simulink model "s20260910_config2torque_sim_chatgpt_multi_torque"  (R2025a)
settings: Solver=daessc  StartTime=0.0  StopTime=20  FixedStep=0.01  MaxStep=0.05  RelTol=1e-3  AbsTol=1e-3  EnableMultiTasking=on
undefined symbols (not defined in the file or in its folder): X, Y, Z
libraries: sm_lib x9, nesl_utility x4, snake_single_module_library_torque x1, slpidlib x1, simulink x1, spsSawtoothGeneratorLib x1, cstblocks x1, snake_single_module_library_torque_multi x1
settings Model: Creator=dperera  LastModifiedBy=dperera
settings SolverCC: AutoScaleAbsTol=off  AlgebraicLoopSolver=TrustRegion  MaxZcPerStep=1.0
settings DataIOCC: LimitDataPoints=on  MaxDataPoints=10000
settings OptimizationCC: ReuseModelBlockBuffer=off  LifeSpan=inf
settings DebuggingCC: UnconnectedInputMsg=warning  UnconnectedOutputMsg=warning  UnconnectedLineMsg=warning  AllowSymbolicDim=off  SubsystemReferenceDiagnosticForUnitTest=warning  SFUnexpectedBacktrackingDiag=warning  SFNoUnconditionalDefaultTransitionDiag=warning  SFExecutionAtInitializationDiag=none  ArithmeticOperatorsInVariantConditions=warning
settings ModelReferenceCC: EnableRefExpFcnMdlSchedulingChecks=on
settings SFSimCC: SimUseLocalCustomCode=off  CustomCodeUndefinedFunction=UseInterfaceOnly
settings RTWCC: RTWUseLocalCustomCode=off  GPUComputeCapability=3.5  DLArmComputeVersion=19.05
settings CodeAppCC: StateflowObjectComments=on
settings GRTTargetCC: TargetLangStandard=C89/C90 (ANSI)
settings ConfigComp: CovMetricSettings=dw  CovSaveCumulativeToWorkspaceVar=on  CovSaveSingleToWorkspaceVar=on  CovExternalEMLEnable=off  CovSFcnEnable=off
settings SimscapeCC: SimscapeLogType=all  SimscapeLogSimulationStatistics=on  SimscapeLogDataHistory=10000.0

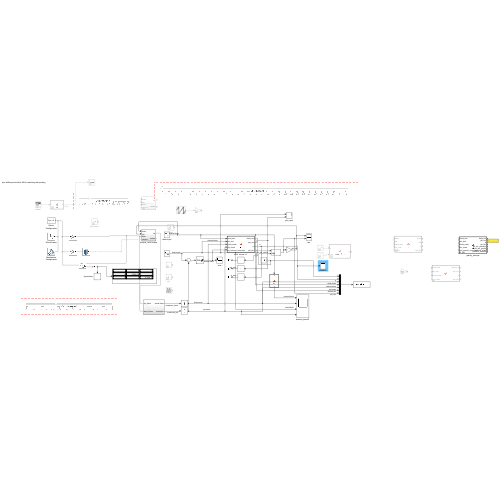
[thumbnail: Simulink's stored preview of the top-level diagram]
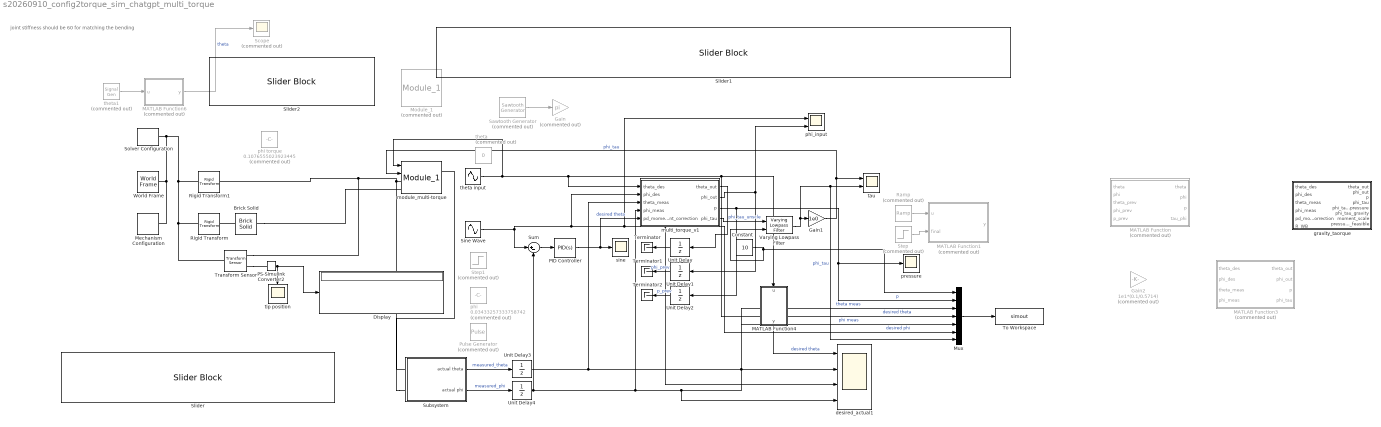
== system s20260910_config2torque_sim_chatgpt_multi_torque ==
  note: joint stiffness should be 60 for matching the bending
  Brick Solid : sm_lib/Body Elements/Brick Solid  BrickDimensions=[0.5 0.5 0.01]  BrickDimensionsUnits=m  ExportEntireGeometry=on  InertiaType=CalculateFromGeometry  BasedOnType=Density  Density=1000  DensityUnits=kg/m^3  Mass=1  MassUnits=kg  CenterOfMass=[0 0 0]  CenterOfMassUnits=m  MomentsOfInertia=[1 1 1]  MomentsOfInertiaUnits=kg*m^2  ProductsOfInertia=[0 0 0]  ProductsOfInertiaUnits=kg*m^2  GraphicType=FromGeometry  MarkerShape=Sphere  MarkerSize=10  GraphicVisPropType=SimpleVisualProperties  GraphicDiffuseColor=[0.5 0.5 0.5]  GraphicOpacity=1  GraphicSpecularColor=[0.5 0.5 0.5 1.0]  GraphicAmbientColor=[0.15 0.15 0.15 1.0]  GraphicEmissiveColor=[0.0 0.0 0.0 1.0]  GraphicShininess=75  DoExposeReferenceFrame=on  SerializedFrames=<Frames/>
  Constant : Constant  Value=10
  Display : Display
  Gain : Gain  Commented=on  Gain=pi
  Gain1 : Gain  Gain=1e0
  Gain2 : Gain  Commented=on  Gain=1e1*(0.1/0.5714)
  MATLAB Function : MATLAB Function  Commented=on  TreatAsAtomicUnit=on
  MATLAB Function1 : MATLAB Function  Commented=on  TreatAsAtomicUnit=on
  MATLAB Function3 : MATLAB Function  Commented=on  TreatAsAtomicUnit=on
  MATLAB Function4 : MATLAB Function  TreatAsAtomicUnit=on
  MATLAB Function6 : MATLAB Function  Commented=on  TreatAsAtomicUnit=on
  Mechanism Configuration : sm_lib/Utilities/Mechanism Configuration  UniformGravity=Constant  GravityVector=[0 0 -9.80665]  GravityVectorUnits=m/s^2  LinearizationDelta=0.001  JointModeTransitionNonlinearIterations=2
  Module_1 : snake_single_module_library_torque/Module_1  Commented=on  SystemSampleTime=-1  VariantActivationTime=update diagram  EmptyChoice=off  PassThrough=off  PassThroughVariantControl=(default)  EmptyChoiceVariantControl=(default)  AllowFlexibleInterface=on  Latency=0  AutoFrameSizeCalculation=off
  Mux : Mux  Inputs=7
  PID Controller : slpidlib/PID Controller  Controller=PID  Form=Parallel  TimeDomain=Continuous-time  UseExternalTs=off  SampleTime=-1  IntegratorMethod=Forward Euler  FilterMethod=Forward Euler  ControllerParametersSource=internal  P=0.3  I=0.1  UseKiTs=off  D=0.0001  UseExternalDerivativeSource=off  N=100  UseFilter=on  TunerSelectOption=Frequency Response Based  InitialConditionSource=internal  InitialConditionForIntegrator=0  InitialConditionForFilter=0  DifferentiatorICPrevScaledInput=0  ExternalReset=none  TrackingMode=off  Kt=1  LimitOutput=on  SatLimitsSource=internal  UpperSaturationLimit=inf  LowerSaturationLimit=-inf  LinearizeAsGain=on  AntiWindupMode=back-calculation  Kb=1  LimitIntegrator=off  UpperIntegratorSaturationLimit=inf  LowerIntegratorSaturationLimit=-inf  POutMin=[]  POutMax=[]  IOutMin=[]  IOutMax=[]  DOutMin=[]  DOutMax=[]  NOutMin=[]  NOutMax=[]  SumOutMin=[]  SumOutMax=[]  SaturationOutMin=[]  SaturationOutMax=[]  PParamMin=[]  PParamMax=[]  IParamMin=[]  IParamMax=[]  DParamMin=[]  DParamMax=[]  NParamMin=[]  NParamMax=[]  KbParamMin=[]  KbParamMax=[]  KtParamMin=[]  KtParamMax=[]  KbOutMin=[]  KbOutMax=[]  KtOutMin=[]  KtOutMax=[]  IntegratorOutMin=[]  IntegratorOutMax=[]  FilterOutMin=[]  FilterOutMax=[]  SumI1OutMin=[]  SumI1OutMax=[]  SumI2OutMin=[]  SumI2OutMax=[]  SumI3OutMin=[]  SumI3OutMax=[]  SumI4OutMin=[]  SumI4OutMax=[]  SumDOutMin=[]  SumDOutMax=[]  DifferentiatorOutMin=[]  DifferentiatorOutMax=[]  FilterDiffOutCoefMin=[]  FilterDiffOutCoefMax=[]  ReciprocalOutMin=[]  ReciprocalOutMax=[]  SumDenOutMin=[]  SumDenOutMax=[]  SumNumOutMin=[]  SumNumOutMax=[]  DivideOutMin=[]  DivideOutMax=[]  UdiffTsProdOutMin=[]  UdiffTsProdOutMax=[]  NTsProdOutMin=[]  NTsProdOutMax=[]  UintegralTsProdOutMin=[]  UintegralTsProdOutMax=[]  UngainTsProdOutMin=[]  UngainTsProdOutMax=[]  ClampingZeroOutDataTypeStr=Inherit: Inherit via back propagation  ClampingZeroOutMin=[]  ClampingZeroOutMax=[]  FilterDenConstantOutDataTypeStr=Inherit: Inherit via back propagation  FilterDenConstantOutMin=[]  FilterDenConstantOutMax=[]  PCopyOutDataTypeStr=Inherit: Inherit via back propagation  PCopyOutMin=[]  PCopyOutMax=[]  NCopyOutDataTypeStr=Inherit: Inherit via back propagation  NCopyOutMin=[]  NCopyOutMax=[]  IntegratorContinuousStateAttributes=''  IntegratorStateMustResolveToSignalObject=off  IntegratorRTWStateStorageClass=Auto  FilterContinuousStateAttributes=''  FilterStateMustResolveToSignalObject=off  FilterRTWStateStorageClass=Auto  ParallelPVariant=InternalParameters  IdealPVariant=Disabled  IVariant=InternalParameters  DVariant=InternalParameters  IntegratorVariant=Continuous  SatVariant=Enabled  AWVariant=BackCalculation  PCopyVariant=Disabled  TRVariant=Disabled  FdbkBlocksVariant=Forward  IdealPFdbkVariant=Disabled  SatFdbkVariant=Disabled  DerivativeFilterVariant=ContFilter  NVariant=InternalParameters  NCopyVariant=Disabled  FilterICVariant=InternalICsFilter  IntegratorICVariant=InternalICs  ExternalResetVariant=Disabled  TRSumVariant=Passthrough  SumFdbkVariant=Disabled  SumVariant=Sum_PID  TsampFilterVariant=InternalTs  TsampNgainVariant=Passthrough  TsampIntegralVariant=Disabled_SignalSpec  ExternalSaturationOutDataTypeStr=Inherit: Same as second input  DerivativeSourceVariant=ErrorSignal  PreIntVariant=InternalPreInt
  PS-Simulink Converter2 : nesl_utility/PS-Simulink Converter  PhysicalDomain=network_engine_domain  SubClassName=ps_output  LeftPortType=input  RightPortType=output  PseudoPeriodic=off  Frequencies=[]  VectorFormat=inherit  Unit=inherit  AffineConversion=off
  Pulse Generator : DiscretePulseGenerator  Commented=on  PulseType=Time based  Amplitude=pi/3  Period=4  PulseWidth=50  PhaseDelay=1
  Ramp : simulink/Sources/Ramp  Commented=on  slope=0.01*2*pi  start=1  InitialOutput=0.001
  Rigid Transform : sm_lib/Frames and Transforms/Rigid Transform  RotationMethod=None  FollAlignAxisA=+X  BaseAlignAxisA=+Y  FollAlignAxisB=+Y  BaseAlignAxisB=+Z  RotationStandardAxis=+Z  RotationAngle=0  RotationAngleUnits=deg  RotationArbitraryAxis=[0 0 1]  RotationSequenceAxes=FollowerAxes  RotationSequence=XYX  RotationSequenceAngles=[0 0 0]  RotationSequenceAnglesUnits=deg  RotationMatrix=[1 0 0;0 1 0;0 0 1]  Quaternion=[1 0 0 0]  TranslationMethod=StandardAxis  TranslationCartesianOffset=[0 0 0]  TranslationCartesianOffsetUnits=m  TranslationStandardAxis=+Z  TranslationStandardOffset=-0.03  TranslationStandardOffsetUnits=m  TranslationROffset=0  TranslationROffsetUnits=m  TranslationThetaOffset=0  TranslationThetaOffsetUnits=deg  TranslationZOffset=0  TranslationZOffsetUnits=m
  Rigid Transform1 : sm_lib/Frames and Transforms/Rigid Transform  RotationMethod=StandardAxis  FollAlignAxisA=+X  BaseAlignAxisA=+Y  FollAlignAxisB=+Y  BaseAlignAxisB=+Z  RotationStandardAxis=+X  RotationAngle=pi/2  RotationAngleUnits=rad  RotationArbitraryAxis=[0 0 1]  RotationSequenceAxes=FollowerAxes  RotationSequence=XYX  RotationSequenceAngles=[0 0 0]  RotationSequenceAnglesUnits=deg  RotationMatrix=[1 0 0;0 1 0;0 0 1]  Quaternion=[1 0 0 0]  TranslationMethod=StandardAxis  TranslationCartesianOffset=[0 0 0]  TranslationCartesianOffsetUnits=m  TranslationStandardAxis=+Z  TranslationStandardOffset=0.5  TranslationStandardOffsetUnits=m  TranslationROffset=0  TranslationROffsetUnits=m  TranslationThetaOffset=0  TranslationThetaOffsetUnits=deg  TranslationZOffset=0  TranslationZOffsetUnits=m
  Sawtooth Generator : spsSawtoothGeneratorLib/Sawtooth Generator  Commented=on  Freq=0.5  Phase=180  Ts=0.001
  Scope : Scope  Commented=on
      settings: ActiveDisplayYMinimum=-3.3334127281449564  ActiveDisplayYMaximum=3.1584952199962761
  Sine Wave : Sin  Amplitude=pi/2-0.3  Bias=pi/2-0.3  Phase=3*pi/2  SampleTime=0
  Slider : SliderBlock  ScaleMin=-3.14  ScaleMax=6
  Slider1 : SliderBlock  ScaleMax=3.14
  Slider2 : SliderBlock  ScaleMax=0.5
  Solver Configuration : nesl_utility/Solver Configuration  PhysicalDomain=network_engine_domain  SubClassName=solver  LeftPortType=input  RightPortType=generic  Tones=[]  Harmonics=[]  SimulateNoise=off  Profile=off  UseLocalSampling=off  EnableSwitchedLinearOptims=on  FrequencyDomain=off  UseCCode=off  RelTol=0.001  AbsTol=1e-06  MinStep=1e-09  ToWorkspace=off  RevertToSquareIcSolve=off  NumHomotopyIterations=100  PhasorMode=off  PhasorModeNumHarmonics=1  ConsistencySolver=NEWTON_XTOL_AFTER_FTOL  IndexReductionMethod=DerivativeReplacement  DoDC=off  ResidualTolerance=1e-09  ConsistencyTolSource=GLOBAL  ConsistencyAbsTol=0.001  ConsistencyRelTol=0.001  ConsistencyTolFactor=0.001  UseLocalSolver=off  LocalSolverChoice=NE_BACKWARD_EULER_ADVANCER  ResolveIndetEquations=on  FunctionEvalNumThread=1  LocalSolverSampleTime=0.001  DoFixedCost=off  MaxNonlinIter=3  MaxModeIter=2  ComputeImpulses=off  ImpulseIterations=2  LinearAlgebra=Sparse  LinearAlgebraNumThread=0  EquationFormulation=NE_TIME_EF  DelaysMemoryBudget=1024  AutomaticFiltering=on  FilteringTimeConstant=0.001  PartitionStorageMethod=AS_NEEDED  PartitionMemoryBudget=1024  PartitionMethod=FAST  MultibodyUseLocalSolver=off  MultibodyLocalSolverChoice=ODE1  MultibodyLocalSolverSampleTime=0.001
  Step : Step  Commented=on  Time=2  SampleTime=0
  Step1 : Step  Commented=on  After=pi/3  SampleTime=0
  Subsystem : Subsystem
  Sum : Sum  Inputs=|+-
  Terminator : Terminator
  Terminator1 : Terminator
  Terminator2 : Terminator
  To Workspace : ToWorkspace  VariableName=simout  SaveFormat=Timeseries  SampleTime=-1
      settings: Save2DSignal=2-D array (concatenate along first dimension)
  Transform Sensor : sm_lib/Frames and Transforms/Transform Sensor  MeasurementFrame=World  RotationSequence=XYX  SenseAngle=off  SenseAxis=off  SenseQ=off  SenseR=on  SenseRotationSequence=off  SenseOmegaX=off  SenseOmegaY=off  SenseOmegaZ=off  SenseOmega=off  SenseQDot=off  SenseRDot=off  SenseRotationSequenceDot=off  SenseAlphaX=off  SenseAlphaY=off  SenseAlphaZ=off  SenseAlpha=off  SenseQDDot=off  SenseRDDot=off  SenseX=off  SenseY=off  SenseZ=off  SenseXYZ=off  SenseRad=off  SenseAzim=off  SenseDist=off  SenseInc=off  SenseXDot=off  SenseYDot=off  SenseZDot=off  SenseXYZDot=off  SenseRadDot=off  SenseAzimDot=off  SenseDistDot=off  SenseIncDot=off  SenseXDDot=off  SenseYDDot=off  SenseZDDot=off  SenseXYZDDot=off  SenseRadDDot=off  SenseAzimDDot=off  SenseDistDDot=off  SenseIncDDot=off
  Unit Delay : UnitDelay  InitialCondition=[0]  SampleTime=-1  HasFrameUpgradeWarning=on
  Unit Delay1 : UnitDelay  InitialCondition=0.0001  SampleTime=-1  HasFrameUpgradeWarning=on
  Unit Delay2 : UnitDelay  InitialCondition=[0.0001;0.01;0.001]  SampleTime=-1  HasFrameUpgradeWarning=on
  Unit Delay3 : UnitDelay  InitialCondition=[0]  SampleTime=-1  HasFrameUpgradeWarning=on
  Unit Delay4 : UnitDelay  InitialCondition=0.0001  SampleTime=-1  HasFrameUpgradeWarning=on
  Varying Lowpass Filter : cstblocks/Linear Parameter Varying/Varying Lowpass Filter  N=1
  World Frame : sm_lib/Frames and Transforms/World Frame
  desired_actual1 : Scope  NumInputPorts=4
      settings: ActiveDisplayYMinimum=-0.37614430678155741  ActiveDisplayYMaximum=3.3852987610340177  DataLoggingVariableName=ScopeData7
  gravity_taorque : MATLAB Function  TreatAsAtomicUnit=on
  module_multi-torque : snake_single_module_library_torque_multi/Module_1  SystemSampleTime=-1  VariantActivationTime=update diagram  EmptyChoice=off  PassThrough=off  PassThroughVariantControl=(default)  EmptyChoiceVariantControl=(default)  AllowFlexibleInterface=on  Latency=0  AutoFrameSizeCalculation=off
  multi_torque_v1 : MATLAB Function  TreatAsAtomicUnit=on
  phi : Constant  Commented=on  Value=0.03433257333758742
  phi torque : Constant  Commented=on  Value=0.1076555023923445
  phi_input : Scope  NumInputPorts=2
      settings: ActiveDisplayYMinimum=-0.36834079509334744  ActiveDisplayYMaximum=3.3160671558401278  DataLoggingVariableName=ScopeData3
  pressure : Scope
      settings: ActiveDisplayYMinimum=-30741.22465781157  ActiveDisplayYMaximum=510004.6447710325  DataLoggingVariableName=ScopeData4
  sine : Scope
      settings: ActiveDisplayYMinimum=-0.41740703510045596  ActiveDisplayYMaximum=3.0703490190244911  DataLoggingVariableName=ScopeData2
  tau : Scope  NumInputPorts=2
      settings: ActiveDisplayYMinimum=-0.07521570426510249  ActiveDisplayYMaximum=0.65254070404289077
  theta : Constant  Commented=on  Value=0
  theta input : Sin  Amplitude=pi-0.1  Frequency=0.1  SampleTime=0
  theta1 : SignalGenerator  Commented=on  WaveForm=sawtooth  Amplitude=pi  Frequency=0.1*2*pi  Units=rad/sec  VectorParams1D=off
  tip position : Scope
      settings: ActiveDisplayYMinimum=-1.2500000000000002  ActiveDisplayYMaximum=1.2500000000000004  DataLoggingVariableName=ScopeData5
  wires:
  Sawtooth Generator/1 -> Gain/1
  theta1/1 -> MATLAB Function6/1(u)
  MATLAB Function6/1(y) -> Scope/1  "theta"
  multi_torque_v1/1(theta_out) -> Unit Delay/1
  multi_torque_v1/2(phi_out) -> Unit Delay1/1, phi_input/2
  multi_torque_v1/3(p) -> Mux/2, pressure/1, Unit Delay2/1  "p"
  theta input/1 -> module_multi-torque/1, multi_torque_v1/1(theta_des), Mux/4, MATLAB Function4/1(u)  "desired theta"
  Ramp/1 -> MATLAB Function1/1(u)
  Step/1 -> MATLAB Function1/2(final)
  MATLAB Function4/1(y) -> desired_actual1/1  "desired theta"
  Gain1/1 -> module_multi-torque/2, tau/1  "phi_tau"
  Sine Wave/1 -> multi_torque_v1/2(phi_des), desired_actual1/3, Mux/6, phi_input/1, Sum/1  "desired phi"
  Subsystem/1(actual theta) -> Unit Delay3/1  "measured_theta"
  Subsystem/2(actual phi) -> Unit Delay4/1  "measured_phi"
  Mux/1 -> To Workspace/1
  PID Controller/1 -> multi_torque_v1/5(pd_moment_correction), sine/1  "desired theta"
  Unit Delay/1 -> Terminator/1
  Unit Delay1/1 -> Terminator1/1  "phi_prev"
  Unit Delay2/1 -> Terminator2/1  "p_prev"
  Unit Delay3/1 -> multi_torque_v1/3(theta_meas), Mux/3, desired_actual1/2  "theta meas"
  Unit Delay4/1 -> multi_torque_v1/4(phi_meas), Mux/5, desired_actual1/4, Sum/2  "phi meas"
  Sum/1 -> PID Controller/1
  multi_torque_v1/4(phi_tau) -> Varying Lowpass Filter/1  "phi_tau_unscle"
  Varying Lowpass Filter/1 -> Mux/7, tau/2, Gain1/1  "phi_tau"
  Constant/1 -> Mux/1, Varying Lowpass Filter/2
  PS-Simulink Converter2/1 -> Display/1, tip position/1
  connections:
  World Frame/RConn1 -- Transform Sensor/LConn1 -- Rigid Transform/LConn1 -- Rigid Transform1/LConn1 -- Solver Configuration/RConn1 -- Mechanism Configuration/RConn1
  Brick Solid/RConn1 -- Rigid Transform/RConn1
  Subsystem/LConn2 -- Transform Sensor/RConn1 -- Rigid Transform1/RConn1 -- module_multi-torque/LConn1
  Brick Solid/LConn1 -- module_multi-torque/LConn2
  Subsystem/LConn1 -- module_multi-torque/RConn1
  Transform Sensor/RConn2 -- PS-Simulink Converter2/LConn1

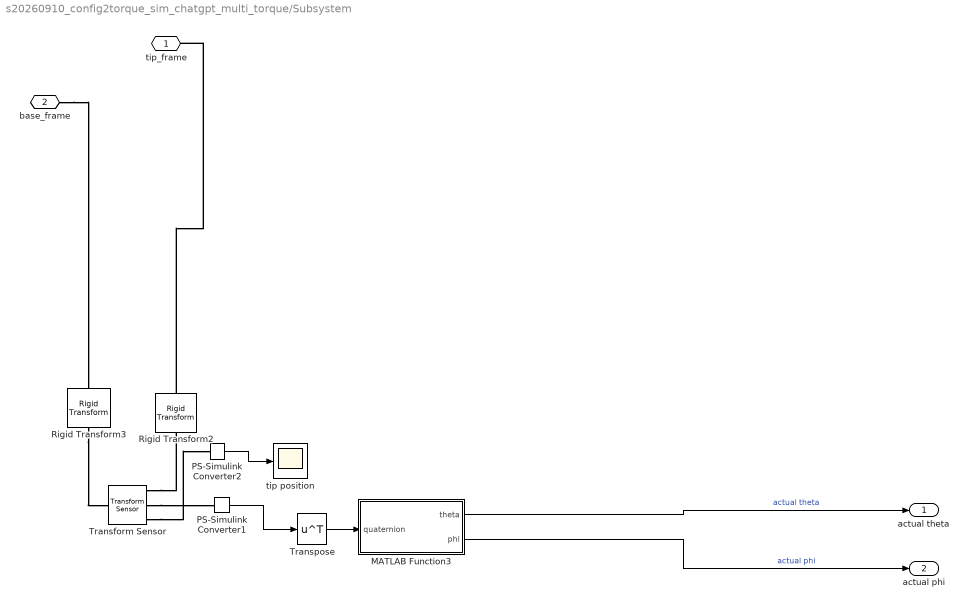
== system s20260910_config2torque_sim_chatgpt_multi_torque/Subsystem ==
  MATLAB Function3 : MATLAB Function  TreatAsAtomicUnit=on
  PS-Simulink Converter1 : nesl_utility/PS-Simulink Converter  PhysicalDomain=network_engine_domain  SubClassName=ps_output  LeftPortType=input  RightPortType=output  PseudoPeriodic=off  Frequencies=[]  VectorFormat=inherit  Unit=inherit  AffineConversion=off
  PS-Simulink Converter2 : nesl_utility/PS-Simulink Converter  PhysicalDomain=network_engine_domain  SubClassName=ps_output  LeftPortType=input  RightPortType=output  PseudoPeriodic=off  Frequencies=[]  VectorFormat=inherit  Unit=inherit  AffineConversion=off
  Rigid Transform2 : sm_lib/Frames and Transforms/Rigid Transform  RotationMethod=RotationSequence  FollAlignAxisA=+X  BaseAlignAxisA=+Y  FollAlignAxisB=+Y  BaseAlignAxisB=+Z  RotationStandardAxis=+Z  RotationAngle=pi  RotationAngleUnits=rad  RotationArbitraryAxis=[0 0 1]  RotationSequenceAxes=FollowerAxes  RotationSequence=XZY  RotationSequenceAngles=[-pi/2 pi 0]  RotationSequenceAnglesUnits=rad  RotationMatrix=[1 0 0;0 1 0;0 0 1]  Quaternion=[1 0 0 0]  TranslationMethod=None  TranslationCartesianOffset=[0 0 0]  TranslationCartesianOffsetUnits=m  TranslationStandardAxis=+Z  TranslationStandardOffset=-0.5  TranslationStandardOffsetUnits=m  TranslationROffset=0  TranslationROffsetUnits=m  TranslationThetaOffset=0  TranslationThetaOffsetUnits=deg  TranslationZOffset=0  TranslationZOffsetUnits=m
  Rigid Transform3 : sm_lib/Frames and Transforms/Rigid Transform  RotationMethod=RotationSequence  FollAlignAxisA=+X  BaseAlignAxisA=+Y  FollAlignAxisB=+Y  BaseAlignAxisB=+Z  RotationStandardAxis=+Z  RotationAngle=pi  RotationAngleUnits=rad  RotationArbitraryAxis=[0 0 1]  RotationSequenceAxes=FollowerAxes  RotationSequence=YXZ  RotationSequenceAngles=[pi -pi/2 0]  RotationSequenceAnglesUnits=rad  RotationMatrix=[1 0 0;0 1 0;0 0 1]  Quaternion=[1 0 0 0]  TranslationMethod=None  TranslationCartesianOffset=[0 0 0]  TranslationCartesianOffsetUnits=m  TranslationStandardAxis=+Z  TranslationStandardOffset=-0.5  TranslationStandardOffsetUnits=m  TranslationROffset=0  TranslationROffsetUnits=m  TranslationThetaOffset=0  TranslationThetaOffsetUnits=deg  TranslationZOffset=0  TranslationZOffsetUnits=m
  Transform Sensor : sm_lib/Frames and Transforms/Transform Sensor  MeasurementFrame=Follower  RotationSequence=XYZ  SenseAngle=off  SenseAxis=off  SenseQ=on  SenseR=off  SenseRotationSequence=off  SenseOmegaX=off  SenseOmegaY=off  SenseOmegaZ=off  SenseOmega=off  SenseQDot=off  SenseRDot=off  SenseRotationSequenceDot=off  SenseAlphaX=off  SenseAlphaY=off  SenseAlphaZ=off  SenseAlpha=off  SenseQDDot=off  SenseRDDot=off  SenseX=off  SenseY=off  SenseZ=off  SenseXYZ=on  SenseRad=off  SenseAzim=off  SenseDist=off  SenseInc=off  SenseXDot=off  SenseYDot=off  SenseZDot=off  SenseXYZDot=off  SenseRadDot=off  SenseAzimDot=off  SenseDistDot=off  SenseIncDot=off  SenseXDDot=off  SenseYDDot=off  SenseZDDot=off  SenseXYZDDot=off  SenseRadDDot=off  SenseAzimDDot=off  SenseDistDDot=off  SenseIncDDot=off
  Transpose : Math  Operator=transpose
  tip position : Scope
      settings: ActiveDisplayYMinimum=-0.036250000065594909  ActiveDisplayYMaximum=0.32625000000729432  DataLoggingVariableName=ScopeData6
  tip_frame : PMIOPort  Side=Left
  base_frame : PMIOPort  Port=2  Side=Left
  actual theta : Outport
  actual phi : Outport  Port=2
  wires:
  PS-Simulink Converter1/1 -> Transpose/1
  Transpose/1 -> MATLAB Function3/1(quaternion)
  MATLAB Function3/2(phi) -> actual phi/1  "actual phi"
  PS-Simulink Converter2/1 -> tip position/1
  MATLAB Function3/1(theta) -> actual theta/1  "actual theta"
  connections:
  Transform Sensor/RConn1 -- Rigid Transform2/RConn1
  Transform Sensor/RConn2 -- PS-Simulink Converter1/LConn1
  Rigid Transform3/RConn1 -- Transform Sensor/LConn1
  Transform Sensor/RConn3 -- PS-Simulink Converter2/LConn1
  base_frame/RConn1 -- Rigid Transform3/LConn1
  Rigid Transform2/LConn1 -- tip_frame/RConn1

== matlab function s20260910_config2torque_sim_chatgpt_multi_torque/MATLAB Function6 ==
  data: u input; y output
function y = fcn(u)

y = wrapToPi(u - pi);

== matlab function s20260910_config2torque_sim_chatgpt_multi_torque/MATLAB Function1 ==
  data: u input; y output; final input
function y = smoothStep(u, final)

y = u*(1-final);

if y <= 0.00001
    y= 0.001;
end

end

== matlab function s20260910_config2torque_sim_chatgpt_multi_torque/MATLAB Function ==
  data: theta input; theta output; phi input; theta_prev input; phi_prev input; p_prev input; phi output; p output; tau_phi output
function [theta, phi, p, tau_phi] = fcn(theta, phi, theta_prev, phi_prev, p_prev)
%#codegen 
% 
% This function computes torque required for the
% 
A = pi * (0.013/2)^2;
r = 0.013;
K = 0.00001;
N = 30;
L = 0.29;
l = L/N;

J_angle = f20260427_3_pressure2config_Jacobian(p_prev, A, K, r);
J_inv = pinv(J_angle);
% p = p_mat(:, i) + J_inv*([theta(i+1); phi(i+1)]-[frw(1,i); frw(2,i)]);
p = p_prev + J_inv*([theta; phi]-[theta_prev; phi_prev]);
% p = m20260427_5_PositivePressures(p);


[f, my, mx, ~, ~] = pressure2force_moment_config(p, A, r, K);
W = [mx; my; 0.0; 0.0; 0.0; f];
J = completeArm_Jacobian(theta_prev, phi_prev, l, N);

tau = J' * W;
tau_phi = tau(2);

== matlab function s20260910_config2torque_sim_chatgpt_multi_torque/gravity_taorque ==
  data: theta_des input; theta_out output; phi_des input; theta_meas input; phi_meas input; phi_out output; p output; phi_tau output; pd_moment_correction input; R_WB input; phi_tau_pressure output; phi_tau_gravity output; moment_scale output; pressure_feasible output
function [theta_out, phi_out, p, phi_tau, ...
          phi_tau_pressure, phi_tau_gravity, ...
          moment_scale, pressure_feasible] = ...
    fcn(theta_des, phi_des, theta_meas, phi_meas, ...
        pd_moment_correction, R_WB)

%#codegen
%
% Inputs:
%   theta_des            : desired bending direction [rad]
%   phi_des              : desired total bending angle [rad]
%   theta_meas           : measured bending direction [rad]
%   phi_meas             : measured total bending angle [rad]
%   pd_moment_correction : PD correction added to bending moment [N*m]
%   R_WB                 : rotation matrix from arm base to world [3x3]
%
%                           v_world = R_WB*v_base
%
% Outputs:
%   theta_out       : desired theta for theta position controller [rad]
%   phi_out         : desired phi for logging [rad]
%   p               : allocated muscle pressures [3x1], Pa
%   phi_tau         : final torque for all 58 phi joints [58x1], N*m
%   phi_tau_pressure: pressure-generated phi-joint torque [58x1], N*m
%   phi_tau_gravity : gravity-compensation torque [58x1], N*m
%   moment_scale    : pressure-allocation moment scaling factor
%   pressure_feasible: true if the requested moment is feasible
%
% phi_tau ordering:
%   phi_tau(1)  = interval 1, Phi1
%   phi_tau(2)  = interval 1, Phi2
%   phi_tau(3)  = interval 2, Phi1
%   phi_tau(4)  = interval 2, Phi2
%   ...
%   phi_tau(57) = interval 29, Phi1
%   phi_tau(58) = interval 29, Phi2

%% Model parameters

A = pi*(0.013/2)^2;     % Effective muscle area [m^2]
r = 0.013;              % Muscle radial offset [m]
K = 0.19223750;         % Continuum bending stiffness [N*m/rad]

N = 29;                 % Number of rigid-link intervals
L = 0.29;               % Arm length [m]
l = L/N;                % Link length [m]

number_phi_joints = 2*N;

% Total module mass is assumed to be 0.100 kg over 30 disks.
% The base disk is fixed but each moving disk retains the same mass.
disk_mass = 0.100/30;   % [kg]

theta_out = theta_des;
phi_out = phi_des;

%% Desired bending moments

% The PD controller modifies the commanded bending moment.
bending_moment_cmd = K*phi_des + pd_moment_correction;

my_des =  bending_moment_cmd*cos(theta_des);
mx_des = -bending_moment_cmd*sin(theta_des);

%% Null-space pressure allocation

Ar = A*r;

% Differential-pressure component. Its sum is zero, so adding a common
% pressure does not change the bending moments.
p_delta = [ ...
    -2*my_des/(3*Ar);
     my_des/(3*Ar) + mx_des/(sqrt(3)*Ar);
     my_des/(3*Ar) - mx_des/(sqrt(3)*Ar)];

p_min = 0;              % Minimum pressure [Pa]
p_max = 350000;         % Maximum pressure: 3.5 bar [Pa]

p_common_min = p_min - min(p_delta);
p_common_max = p_max - max(p_delta);

if p_common_min <= p_common_max

    % Requested bending moment is feasible.
    p_common = 0.5*(p_common_min + p_common_max);

    p = p_delta + p_common;

    moment_scale = 1.0;
    pressure_feasible = true;

else

    % Scale the differential pressures while preserving theta.
    pressure_span = max(p_delta) - min(p_delta);

    if pressure_span > 1e-12
        moment_scale = (p_max - p_min)/pressure_span;
    else
        moment_scale = 1.0;
    end

    p_delta = moment_scale*p_delta;

    p_common_min = p_min - min(p_delta);
    p_common_max = p_max - max(p_delta);

    p_common = 0.5*(p_common_min + p_common_max);

    p = p_delta + p_common;

    pressure_feasible = false;

end

%% Recalculate the achievable moments

moment_y = -(A*r*(-p(2) - p(3) + 2*p(1)))/2;
moment_x =  A*r*sqrt(3)*(p(2) - p(3))/2;

%% Moment-only tip wrench

% Wrench convention:
% [Mx; My; Mz; Fx; Fy; Fz]
%
% The axial force is intentionally excluded.
W_pressure = [moment_x;
              moment_y;
              0;
              0;
              0;
              0];

%% Select the configuration used by the Jacobian and gravity model

% Theta is undefined when the arm is straight. Use commanded theta in
% this small region.
if abs(phi_meas) < 1e-6
    theta_for_J = theta_des;
else
    theta_for_J = theta_meas;
end

phi_for_J = phi_meas;

%% Pressure-generated joint torques

J_tip = completeArm_Jacobian( ...
    theta_for_J, phi_for_J, l, N);

tau_pressure_all = J_tip.'*W_pressure;

phi_tau_pressure = zeros(number_phi_joints,1);

for interval = 1:N

    % Columns in the complete 4N-joint Jacobian
    index_all_phi1 = 4*(interval-1) + 2;
    index_all_phi2 = 4*(interval-1) + 3;

    % Locations in the 2N-element output vector
    index_phi1 = 2*interval - 1;
    index_phi2 = 2*interval;

    phi_tau_pressure(index_phi1) = ...
        tau_pressure_all(index_all_phi1);

    phi_tau_pressure(index_phi2) = ...
        tau_pressure_all(index_all_phi2);
end

%% Convert world gravity into the arm-base frame

gravity_world = [0;
                 0;
                -9.80665];

% R_WB maps base-frame vectors into the world frame.
% Therefore, its transpose maps world vectors into the base frame.
gravity_base = R_WB.'*gravity_world;

gravity_force_disk = disk_mass*gravity_base;

%% Rotation matrices for one rigid-link interval

alpha = phi_for_J/(2*N);

ct = cos(theta_for_J);
st = sin(theta_for_J);

ca = cos(alpha);
sa = sin(alpha);

Rz_theta = [ct, -st, 0;
            st,  ct, 0;
             0,   0, 1];

Rz_minus_theta = [ ct, st, 0;
                   -st, ct, 0;
                     0,  0, 1];

Ry_alpha = [ ca, 0, sa;
              0, 1,  0;
            -sa, 0, ca];

%% Joint axes, joint positions and disk COM positions

joint_axis = zeros(3,number_phi_joints);
joint_position = zeros(3,number_phi_joints);
disk_position = zeros(3,N);

% Pose at the base of the current interval
R_current = eye(3);
position_current = zeros(3,1);

translation_local = [0; 0; l];

for interval = 1:N

    index_phi1 = 2*interval - 1;
    index_phi2 = 2*interval;

    % Apply Rz(theta).
    R_after_theta = R_current*Rz_theta;

    % First phi joint is located at the proximal disk.
    joint_axis(:,index_phi1) = R_after_theta(:,2);
    joint_position(:,index_phi1) = position_current;

    % Apply the first Ry(alpha).
    R_after_phi1 = R_after_theta*Ry_alpha;

    % Translate to the next disk.
    next_disk_position = ...
        position_current + R_after_phi1*translation_local;

    % Second phi joint is located at the distal disk.
    joint_axis(:,index_phi2) = R_after_phi1(:,2);
    joint_position(:,index_phi2) = next_disk_position;

    % Assumption: the disk COM is at the disk-frame origin.
    disk_position(:,interval) = next_disk_position;

    % Complete the interval:
    % Ry(alpha), followed by Rz(-theta).
    R_current = ...
        R_after_phi1*Ry_alpha*Rz_minus_theta;

    position_current = next_disk_position;
end

%% Accumulate downstream gravity forces and moments

% downstream_force(:,i) contains the total gravity force from disk i
% through disk N.
%
% downstream_moment_origin(:,i) contains their total gravity moment
% calculated about the arm-base origin.

downstream_force = zeros(3,N+1);
downstream_moment_origin = zeros(3,N+1);

for disk_number = N:-1:1

    downstream_force(:,disk_number) = ...
        downstream_force(:,disk_number+1) + ...
        gravity_force_disk;

    downstream_moment_origin(:,disk_number) = ...
        downstream_moment_origin(:,disk_number+1) + ...
        cross(disk_position(:,disk_number), ...
              gravity_force_disk);
end

%% Calculate gravity torque at all 58 phi joints

phi_tau_gravity_load = zeros(number_phi_joints,1);

for interval = 1:N

    index_phi1 = 2*interval - 1;
    index_phi2 = 2*interval;

    force_downstream = downstream_force(:,interval);
    moment_downstream_origin = ...
        downstream_moment_origin(:,interval);

    % Gravity moment about the first phi joint
    moment_about_phi1 = ...
        moment_downstream_origin ...
        - cross(joint_position(:,index_phi1), ...
                force_downstream);

    phi_tau_gravity_load(index_phi1) = ...
        joint_axis(:,index_phi1).'*moment_about_phi1;

    % Gravity moment about the second phi joint
    moment_about_phi2 = ...
        moment_downstream_origin ...
        - cross(joint_position(:,index_phi2), ...
                force_downstream);

    phi_tau_gravity_load(index_phi2) = ...
        joint_axis(:,index_phi2).'*moment_about_phi2;
end

%% Gravity compensation

% Gravity compensation acts opposite to the gravity-generated load.
phi_tau_gravity = -phi_tau_gravity_load;

%% Final joint torque commands

% pd_moment_correction is already included in the pressure-generated
% moment. Do not add the same PD output again elsewhere.
phi_tau = phi_tau_pressure + phi_tau_gravity;

end

== matlab function s20260910_config2torque_sim_chatgpt_multi_torque/Subsystem/MATLAB Function3 ==
  data: quaternion input; theta output; phi output
function [theta, phi] = IMU2Config(quaternion)
%#codegen
T = quat2rotm(quaternion);

theta= wrapToPi(atan2(T(2,3),T(1,3)));
phi= (acos(T(3,3)));

end

== matlab function s20260910_config2torque_sim_chatgpt_multi_torque/MATLAB Function4 ==
  data: u input; y output
function y = fcn(u)
%$codegen
y = wrapToPi(u);

== matlab function s20260910_config2torque_sim_chatgpt_multi_torque/MATLAB Function3 ==
  data: theta_des input; theta_out output; phi_des input; theta_meas input; phi_meas input; phi_out output; p output; phi_tau output
function [theta_out, phi_out, p, phi_tau] = ...
    fcn(theta_des, phi_des, theta_meas, phi_meas)

%#codegen
%
% Inputs:
%   theta_des  : desired bending direction [rad]
%   phi_des    : desired total bending angle [rad]
%   theta_meas : measured bending direction [rad]
%   phi_meas   : measured total bending angle [rad]
%
% Outputs:
%   theta_out  : desired theta passed to the theta position controller
%   phi_out    : desired phi for logging
%   p          : calculated muscle pressures [Pa]
%   tau_phi    : first phi-joint torque [N*m]

%% Model parameters

A = pi*(0.013/2)^2;     % Muscle area [m^2]
r = 0.013;              % Muscle radial offset [m]
K = 0.19223750;            % Continuum bending stiffness [N*m/rad]

N = 29;                 % Number of rigid-link intervals
L = 0.29;               % Arm length [m]
l = L/N;                % Link length [m]

theta_out = theta_des;
phi_out = phi_des;

%% Select the common pressure

% Maximum expected bending angle
phi_max = pi;

% Minimum common pressure required to prevent negative pressures.
% The factor 1.10 adds a 10% margin.
p_common = 1.10*(2*K*phi_max)/(3*A*r);

%% Direct configuration-to-pressure mapping

% Desired bending moments
my_des = K*phi_des*cos(theta_des);
mx_des = -K*phi_des*sin(theta_des);

Ar = A*r;

p1 = p_common - 2*my_des/(3*Ar);

p2 = p_common ...
   + my_des/(3*Ar) ...
   + mx_des/(sqrt(3)*Ar);

p3 = p_common ...
   + my_des/(3*Ar) ...
   - mx_des/(sqrt(3)*Ar);

p = [p1; p2; p3];

% Numerical protection. Adding the same pressure to all three muscles
% does not change the desired bending moments.
% minimum_pressure = min(p);
% 
% if minimum_pressure < 0
%     p = p - minimum_pressure;
% end

%% Calculate the tip wrench

% Corrected axial force
force_z = A*sum(p);

% Recalculate moments from the resulting pressures
moment_y = -(A*r*(-p(2) - p(3) + 2*p(1)))/2;
moment_x = A*r*sqrt(3)*(p(2) - p(3))/2;

% Tip-frame wrench:
% [Mx; My; Mz; Fx; Fy; Fz]
W = [moment_x;
     moment_y;
     0;
     0;
     0;
     0];

%% Calculate joint torques at the measured configuration

% Theta from a tip-pose estimator may be undefined when phi is almost zero.
% In that small region, use the commanded theta.
if abs(phi_meas) < 1e-6
    theta_for_J = theta_des;
else
    theta_for_J = theta_meas;
end

J = completeArm_Jacobian( ...
    theta_for_J, phi_meas, l, N);

tau = J.'*W;

% First phi joint. This preserves your current common-torque experiment.
phi_tau = tau(2);

end

== matlab function s20260910_config2torque_sim_chatgpt_multi_torque/multi_torque_v1 ==
  data: theta_des input; theta_out output; phi_des input; theta_meas input; phi_meas input; phi_out output; p output; phi_tau output; pd_moment_correction input
function [theta_out, phi_out, p, phi_tau] = ...
    fcn(theta_des, phi_des, theta_meas, phi_meas, pd_moment_correction)

%#codegen
%
% Inputs:
%   theta_des  : desired bending direction [rad]
%   phi_des    : desired total bending angle [rad]
%   theta_meas : measured bending direction [rad]
%   phi_meas   : measured total bending angle [rad]
%
% Outputs:
%   theta_out  : desired theta passed to the theta position controller
%   phi_out    : desired phi for logging
%   p          : calculated muscle pressures [Pa]
%   tau_phi    : first phi-joint torque [N*m]

%% Model parameters

A = pi*(0.013/2)^2;     % Muscle area [m^2]
r = 0.013;              % Muscle radial offset [m]
K = 0.19223750;            % Continuum bending stiffness [N*m/rad]

N = 29;                 % Number of rigid-link intervals
L = 0.29;               % Arm length [m]
l = L/N;                % Link length [m]

theta_out = theta_des;
phi_out = phi_des;


%% Desired bending moments

% my_des = K*phi_des*cos(theta_des);
% mx_des = -K*phi_des*sin(theta_des);

bending_moment_cmd = ...
    K*phi_des + pd_moment_correction;

my_des = bending_moment_cmd*cos(theta_des);
mx_des = -bending_moment_cmd*sin(theta_des);

%% Null-space pressure allocation

Ar = A*r;

% Differential pressures producing the desired moments.
% Their sum is zero.
p_delta = [ ...
    -2*my_des/(3*Ar);
     my_des/(3*Ar) + mx_des/(sqrt(3)*Ar);
     my_des/(3*Ar) - mx_des/(sqrt(3)*Ar)];

% Physical pressure limits
p_min = 0;          % [Pa]
p_max = 350000;     % 3.5 bar [Pa]

% Range of common pressure that satisfies all pressure limits
p_common_min = p_min - min(p_delta);
p_common_max = p_max - max(p_delta);

if p_common_min <= p_common_max

    % Desired bending moment is feasible.
    % Midpoint gives equal margin from the upper and lower limits.
    p_common = 0.5*(p_common_min + p_common_max);

    p = p_delta + p_common;

    moment_scale = 1.0;
    pressure_feasible = true;

else

    % Requested moment cannot be generated within the pressure limits.
    % Scale the differential pressures while preserving theta.
    pressure_span = max(p_delta) - min(p_delta);

    if pressure_span > 1e-12
        moment_scale = (p_max - p_min)/pressure_span;
    else
        moment_scale = 1.0;
    end

    p_delta = moment_scale*p_delta;

    % Recalculate the feasible common-pressure interval
    p_common_min = p_min - min(p_delta);
    p_common_max = p_max - max(p_delta);

    p_common = 0.5*(p_common_min + p_common_max);

    p = p_delta + p_common;

    pressure_feasible = false;

end

%% Recalculate achievable moments from allocated pressures

moment_y = -(A*r*(-p(2) - p(3) + 2*p(1)))/2;
moment_x = A*r*sqrt(3)*(p(2) - p(3))/2;

%% Moment-only tip wrench

W = [moment_x;
     moment_y;
     0;
     0;
     0;
     0];

%% Joint torque calculation

if abs(phi_meas) < 1e-6
    theta_for_J = theta_des;
else
    theta_for_J = theta_meas;
end

J = completeArm_Jacobian( ...
    theta_for_J, phi_meas, l, N);

tau = J.'*W;

ii = 1:1:N;
idx = 2+4*(ii-1);

phi_tau = tau(idx);

end
